simulink model "PMSM_FOC"  (R2024b)
settings: Solver=FixedStepAuto  StartTime=0.0  StopTime=0.3  FixedStep=2e-7  MaxStep=1e-6  RelTol=1e-3
model workspace (MAT data in the model file):
  Kr = 5
  Wc = 10
undefined symbols (not defined in the file): bm, J, Ld, Lq, P, Rs
libraries: simulink x2, spsDCVoltageSourceLib x1, spsMeanLib x1, slpidlib x1, spsPermanentMagnetSynchronousMachineLib x1, spsUniversalBridgeLib x1, sps_lib x1
settings Model: Creator=t'c  LastModifiedBy=t'c

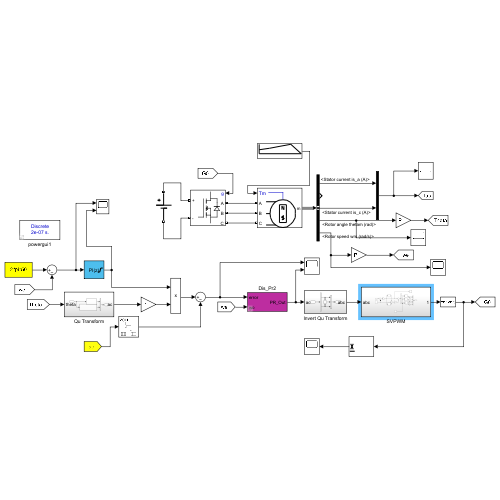
[thumbnail: Simulink's stored preview of the top-level diagram]
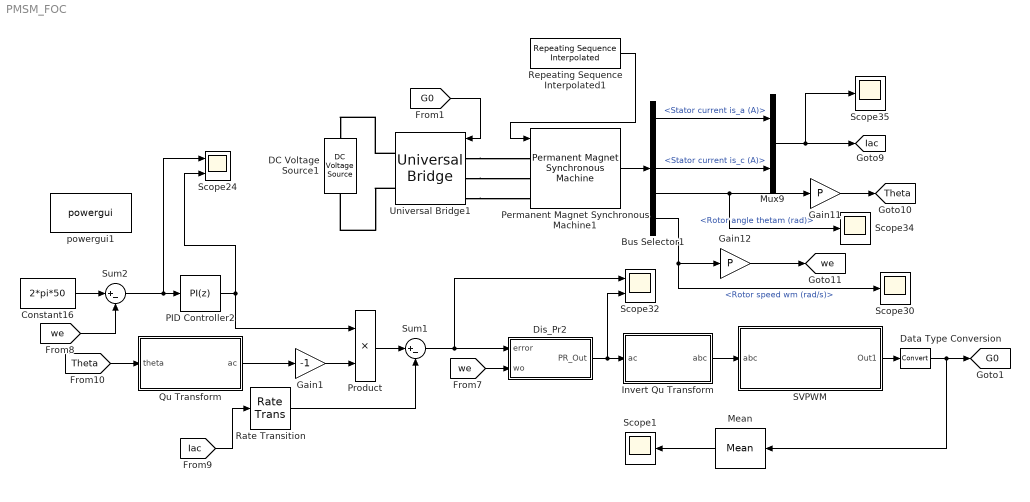
== system PMSM_FOC ==
  Bus Selector1 : BusSelector  OutputSignals=Stator current is_a (A),Stator current is_b (A),Stator current is_c (A),Rotor angle thetam (rad),Rotor speed wm (rad/s)
  Constant16 : Constant  Value=2*pi*50
  DC Voltage Source1 : spsDCVoltageSourceLib/DC Voltage Source  Amplitude=600  Measurements=None
  Data Type Conversion : DataTypeConversion  SaturateOnIntegerOverflow=off  RndMeth=Floor
  Dis_Pr2 : Subsystem  mask{Ts=5e-5, Kp=1, Kr=30, Wc=60}
      mask DialogControl pa Prompt: 参数
  Gain1 : Gain  Gain=-1
  Gain11 : Gain  Gain=P
  Gain12 : Gain  Gain=P
  Invert Qu Transform : Subsystem
  Mean : spsMeanLib/Mean  Freq=20000  Vinit=0  Ts=0
  Mux9 : Mux  Inputs=2
  PID Controller2 : slpidlib/PID Controller  Controller=PI  Form=Parallel  TimeDomain=Discrete-time  UseExternalTs=off  SampleTime=-1  IntegratorMethod=Forward Euler  FilterMethod=Forward Euler  ControllerParametersSource=internal  P=0.02  I=10  UseKiTs=off  D=0  UseExternalDerivativeSource=off  N=100  UseFilter=on  TunerSelectOption=Transfer Function Based (PID Tuner App)  InitialConditionSource=internal  InitialConditionForIntegrator=0  InitialConditionForFilter=0  DifferentiatorICPrevScaledInput=0  ExternalReset=none  TrackingMode=off  Kt=1  LimitOutput=on  SatLimitsSource=internal  UpperSaturationLimit=100  LowerSaturationLimit=-100  LinearizeAsGain=on  AntiWindupMode=none  Kb=1  LimitIntegrator=off  UpperIntegratorSaturationLimit=inf  LowerIntegratorSaturationLimit=-inf  POutMin=[]  POutMax=[]  IOutMin=[]  IOutMax=[]  DOutMin=[]  DOutMax=[]  NOutMin=[]  NOutMax=[]  SumOutMin=[]  SumOutMax=[]  SaturationOutMin=[]  SaturationOutMax=[]  PParamMin=[]  PParamMax=[]  IParamMin=[]  IParamMax=[]  DParamMin=[]  DParamMax=[]  NParamMin=[]  NParamMax=[]  KbParamMin=[]  KbParamMax=[]  KtParamMin=[]  KtParamMax=[]  KbOutMin=[]  KbOutMax=[]  KtOutMin=[]  KtOutMax=[]  IntegratorOutMin=[]  IntegratorOutMax=[]  FilterOutMin=[]  FilterOutMax=[]  SumI1OutMin=[]  SumI1OutMax=[]  SumI2OutMin=[]  SumI2OutMax=[]  SumI3OutMin=[]  SumI3OutMax=[]  SumI4OutMin=[]  SumI4OutMax=[]  SumDOutMin=[]  SumDOutMax=[]  DifferentiatorOutMin=[]  DifferentiatorOutMax=[]  FilterDiffOutCoefMin=[]  FilterDiffOutCoefMax=[]  ReciprocalOutMin=[]  ReciprocalOutMax=[]  SumDenOutMin=[]  SumDenOutMax=[]  SumNumOutMin=[]  SumNumOutMax=[]  DivideOutMin=[]  DivideOutMax=[]  UdiffTsProdOutMin=[]  UdiffTsProdOutMax=[]  NTsProdOutMin=[]  NTsProdOutMax=[]  UintegralTsProdOutMin=[]  UintegralTsProdOutMax=[]  UngainTsProdOutMin=[]  UngainTsProdOutMax=[]  ClampingZeroOutDataTypeStr=Inherit: Inherit via back propagation  ClampingZeroOutMin=[]  ClampingZeroOutMax=[]  FilterDenConstantOutDataTypeStr=Inherit: Inherit via back propagation  FilterDenConstantOutMin=[]  FilterDenConstantOutMax=[]  PCopyOutDataTypeStr=Inherit: Inherit via back propagation  PCopyOutMin=[]  PCopyOutMax=[]  NCopyOutDataTypeStr=Inherit: Inherit via back propagation  NCopyOutMin=[]  NCopyOutMax=[]  IntegratorContinuousStateAttributes=''  IntegratorStateMustResolveToSignalObject=off  IntegratorRTWStateStorageClass=Auto  FilterContinuousStateAttributes=''  FilterStateMustResolveToSignalObject=off  FilterRTWStateStorageClass=Auto  ParallelPVariant=InternalParameters  IdealPVariant=Disabled  IVariant=InternalParameters  DVariant=Disabled  IntegratorVariant=Discrete  SatVariant=Enabled  AWVariant=Passthrough  PCopyVariant=Disabled  TRVariant=Disabled  FdbkBlocksVariant=Forward  IdealPFdbkVariant=Disabled  SatFdbkVariant=Disabled  DerivativeFilterVariant=Disabled  NVariant=Disabled  NCopyVariant=Disabled_SignalSpec  FilterICVariant=Disabled  IntegratorICVariant=InternalICs  ExternalResetVariant=Disabled  TRSumVariant=Passthrough  SumFdbkVariant=Disabled  SumVariant=Sum_PI  TsampFilterVariant=InternalTs  TsampNgainVariant=Passthrough  TsampIntegralVariant=Disabled_SignalSpec  ExternalSaturationOutDataTypeStr=Inherit: Same as second input  DerivativeSourceVariant=Disabled  PreIntVariant=InternalPreInt
  Permanent Magnet Synchronous Machine1 : spsPermanentMagnetSynchronousMachineLib/Permanent Magnet Synchronous Machine  NbPhases=3  FluxDistribution=Sinusoidal  RotorType=Salient-pole  MechanicalLoad=Torque Tm  PresetModel=No  ShowDetailedParameters=on  MeasurementBus=off  Resistance=Rs  Inductance=8.5e-3  dqInductances=[Ld,Lq]  La=0.000395  MachineConstant=Flux linkage established by magnets (V.s)  Flux=flux  VoltageCst=98.6707  TorqueCst=0.816  Flat=120  Mechanical=[J bm P 0]  PolePairs=4  InitialConditions=[0,0, 0,0]  InitialConditions5ph=[0 0 0 0 0 0]  RefAngle=Aligned with phase A axis (original Park)  IterativeDiscreteModel=Trapezoidal non iterative  TsBlock=-1  TsPowergui=0
  Product : Product
  Qu Transform : Subsystem
  Rate Transition : RateTransition  OutPortSampleTime=5e-5
  Repeating Sequence Interpolated1 : simulink/Sources/Repeating Sequence Interpolated  OutValues=[0.2 0.3 0.4 0.5 0].'  TimeValues=[0 0.1 0.2 0.3 0.4 ].'  LookUpMeth=Use Input Below  tsamp=1e-1  OutMin=[]  OutMax=[]  OutDataTypeStr=double  OutputDataTypeScalingMode=double  OutDataType=fixdt(0,8)  OutScaling=2^-10
  SVPWM : Subsystem
  Scope{1,30,34..35} (4 alike) : Scope
  Scope24 : Scope  NumInputPorts=2
  Scope32 : Scope  NumInputPorts=2
  Sum1 : Sum  Inputs=|+-
  Sum2 : Sum  Inputs=|+-
  Universal Bridge1 : spsUniversalBridgeLib/Universal Bridge  Arms=3  SnubberResistance=1e5  SnubberCapacitance=inf  Device=MOSFET / Diodes  Ron=1e-3  Lon=0  ForwardVoltages="[  0  0  ]"  ForwardVoltage=0  GTOparameters=[ 10e-6 , 20e-6 ]  IGBTparameters=[ 1e-6 , 2e-6 ]  Measurements=None  Measurements_2=None  converterType=Rectifier
  powergui1 : sps_lib/powergui  Priority=1  SimulationMode=Discrete  SampleTime=2e-7  frequency=60  Iterations=50  frequencyindice=0  Pbase=100e6  ErrMax=1e-4  UnitsV=kV  UnitsW=MW  buscounter=0  FunctionMessages=off  echomessages=off  EnableUseOfTLC=off  CurrentSourceSwitches=off  DisableSnubberDevices=off  DisableRonSwitches=off  DisableVfSwitches=off  DisplayEquations=off  AutomaticDiscreteSolvers=off  SolverType=Tustin/Backward Euler (TBE)  Interpol=off  ExternalGateDelay=off  methode=off  Ts=100  x0status=blocks  SPID=on  SwTol=0  HookPort=off  NonlinearTolerance=1e-4  nMaxIteration=100  ContinueOnMaxIteration=off  RestoreLinks=warning  ResistiveCurrentMeasurement=off  Frange=[0:2:500]  Ylog=off  Xlog=on  ShowGrid=off  save=off  variable=ZData  structure=0  ZoomFFT=off  StartTime=0.0  cycles=1  DisplayStyle=1  fundamental=60  FreqAxis=off  MaxFrequency=1000  frequencyindicesteady=1  RmsSteady=1  display=off
  tag scope: G0=global, Iac=global, Theta=global, we=global
  wires:
  Repeating Sequence Interpolated1/1 -> Permanent Magnet Synchronous Machine1/1
  Sum1/1 -> Dis_Pr2/1(error), Scope32/1
  Gain12/1 -> [we]
  Gain11/1 -> [Theta]
  PID Controller2/1 -> Scope24/2, Product/1
  [we] -> Dis_Pr2/2(wo)
  Constant16/1 -> Sum2/1
  Sum2/1 -> Scope24/1, PID Controller2/1
  Mux9/1 -> [Iac], Scope35/1
  Bus Selector1/1 -> Mux9/1  "<Stator current is_a (A)>"
  Bus Selector1/4 -> Gain11/1, Scope34/1  "<Rotor angle thetam (rad)>"
  Bus Selector1/5 -> Gain12/1, Scope30/1  "<Rotor speed wm (rad/s)>"
  Permanent Magnet Synchronous Machine1/1 -> Bus Selector1/1
  Bus Selector1/3 -> Mux9/2  "<Stator current is_c (A)>"
  Dis_Pr2/1(PR_Out) -> Scope32/2, Invert Qu Transform/1(ac)
  Product/1 -> Sum1/1
  [we] -> Sum2/2
  [Iac] -> Rate Transition/1
  [G0] -> Universal Bridge1/1
  [Theta] -> Qu Transform/1(theta)
  Qu Transform/1(ac) -> Gain1/1
  Gain1/1 -> Product/2
  Mean/1 -> Scope1/1
  SVPWM/1(Out1) -> Data Type Conversion/1
  Data Type Conversion/1 -> [G0], Mean/1
  Invert Qu Transform/1(abc) -> SVPWM/1(abc)
  Rate Transition/1 -> Sum1/2
  connections:
  Universal Bridge1/LConn2 -- Permanent Magnet Synchronous Machine1/LConn2
  Universal Bridge1/LConn1 -- Permanent Magnet Synchronous Machine1/LConn1
  Universal Bridge1/RConn2 -- DC Voltage Source1/LConn1
  Universal Bridge1/RConn1 -- DC Voltage Source1/RConn1
  Universal Bridge1/LConn3 -- Permanent Magnet Synchronous Machine1/LConn3

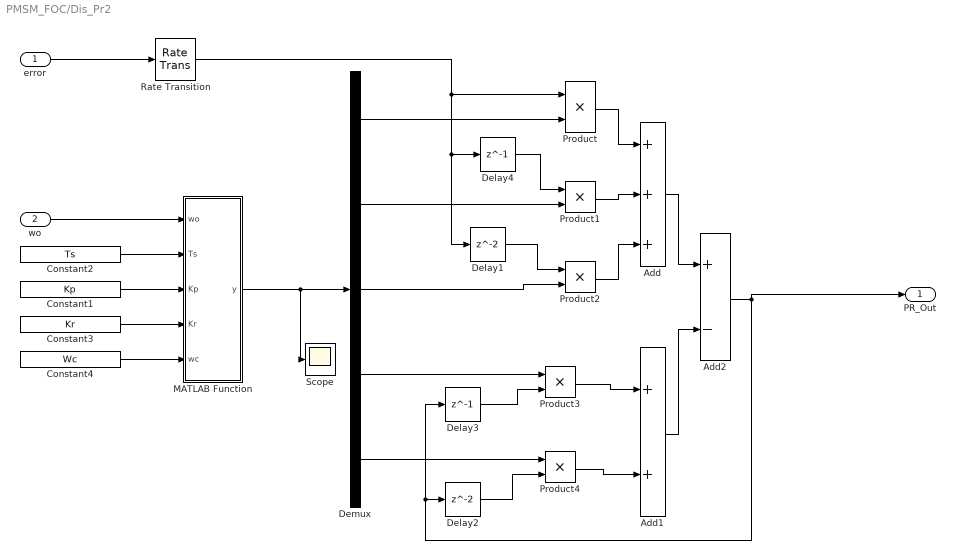
== system PMSM_FOC/Dis_Pr2 ==
  error : Inport
  wo : Inport  Port=2
  Add : Sum  Inputs=+++
  Add1 : Sum
  Add2 : Sum  Inputs=+-
  Constant1 : Constant  Value=Kp  SampleTime=-1
  Constant2 : Constant  Value=Ts  SampleTime=-1
  Constant3 : Constant  Value=Kr  SampleTime=-1
  Constant4 : Constant  Value=Wc  SampleTime=-1
  Delay1 : Delay  SampleTime=5e-5
  Delay2 : Delay  SampleTime=5e-5
  Delay3 : Delay  DelayLength=1  SampleTime=5e-5
  Delay4 : Delay  DelayLength=1  SampleTime=5e-5
  Demux : Demux  Outputs=5
  MATLAB Function : MATLAB Function  TreatAsAtomicUnit=on
  Product{,1..4} (5 alike) : Product
  Rate Transition : RateTransition  OutPortSampleTimeOpt=Inherit  OutPortSampleTime=5e-5
  Scope : Scope
  PR_Out : Outport
  wires:
  Rate Transition/1 -> Product/1, Delay4/1, Delay1/1
  Add2/1 -> PR_Out/1, Delay3/1, Delay2/1
  error/1 -> Rate Transition/1
  Constant4/1 -> MATLAB Function/5(wc)
  Constant3/1 -> MATLAB Function/4(Kr)
  Constant1/1 -> MATLAB Function/3(Kp)
  Constant2/1 -> MATLAB Function/2(Ts)
  Demux/3 -> Product2/2
  Delay1/1 -> Product2/1
  Demux/2 -> Product1/2
  Delay4/1 -> Product1/1
  Product/1 -> Add/1
  Product1/1 -> Add/2
  Product2/1 -> Add/3
  Product3/1 -> Add1/1
  Product4/1 -> Add1/2
  Add/1 -> Add2/1
  Add1/1 -> Add2/2
  Delay2/1 -> Product4/2
  wo/1 -> MATLAB Function/1(wo)
  Delay3/1 -> Product3/2
  Demux/4 -> Product3/1
  Demux/5 -> Product4/1
  Demux/1 -> Product/2
  MATLAB Function/1(y) -> Demux/1, Scope/1

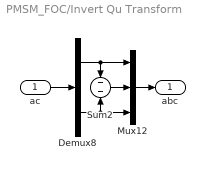
== system PMSM_FOC/Invert Qu Transform ==
  ac : Inport
  Demux8 : Demux  Outputs=2
  Mux12 : Mux  Inputs=3
  Sum2 : Sum  Inputs=-|-
  abc : Outport
  wires:
  Demux8/1 -> Mux12/1, Sum2/1
  ac/1 -> Demux8/1
  Sum2/1 -> Mux12/2
  Demux8/2 -> Mux12/3, Sum2/2
  Mux12/1 -> abc/1

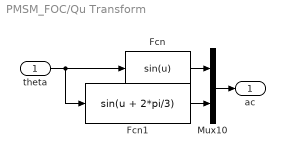
== system PMSM_FOC/Qu Transform ==
  theta : Inport
  Fcn : Fcn  Expr=sin(u)
  Fcn1 : Fcn  Expr=sin(u + 2*pi/3)
  Mux10 : Mux  Inputs=2
  ac : Outport
  wires:
  Mux10/1 -> ac/1
  Fcn/1 -> Mux10/1
  Fcn1/1 -> Mux10/2
  theta/1 -> Fcn1/1, Fcn/1

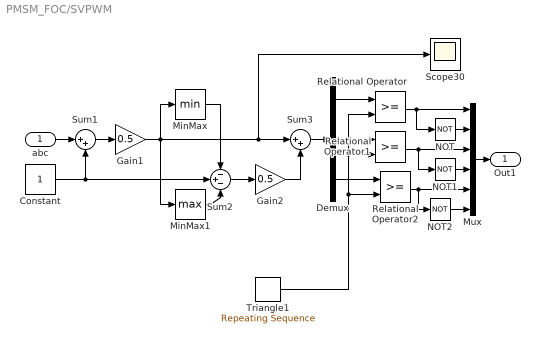
== system PMSM_FOC/SVPWM ==
  abc : Inport
  Constant : Constant
  Demux : Demux  Outputs=3
  Gain1 : Gain  Gain=0.5
  Gain2 : Gain  Gain=0.5
  MinMax : MinMax
  MinMax1 : MinMax  Function=max
  Mux : Mux  Inputs=6
  NOT : Logic  Operator=NOT  IconShape=distinctive  AllPortsSameDT=off  OutDataTypeStr=boolean
  NOT1 : Logic  Operator=NOT  IconShape=distinctive  AllPortsSameDT=off  OutDataTypeStr=boolean
  NOT2 : Logic  Operator=NOT  IconShape=distinctive  AllPortsSameDT=off  OutDataTypeStr=boolean
  Relational Operator : RelationalOperator  OutDataTypeStr=boolean  RndMeth=Simplest  InputSameDT=off
  Relational Operator1 : RelationalOperator  OutDataTypeStr=boolean  RndMeth=Simplest  InputSameDT=off
  Relational Operator2 : RelationalOperator  OutDataTypeStr=boolean  RndMeth=Simplest  InputSameDT=off
  Scope30 : Scope
  Sum1 : Sum  Inputs=|++
  Sum2 : Sum  Inputs=-+-
  Sum3 : Sum  Inputs=|++
  Triangle1 : simulink/Sources/Repeating Sequence  rep_seq_t=[0 1/20000/2 1/20000]  rep_seq_y=[0 1 0]
  Out1 : Outport
  wires:
  abc/1 -> Sum1/1
  Sum1/1 -> Gain1/1
  Constant/1 -> Sum1/2, Sum2/2
  MinMax/1 -> Sum2/1
  Gain1/1 -> Scope30/1, Sum3/1, MinMax1/1, MinMax/1
  MinMax1/1 -> Sum2/3
  Sum2/1 -> Gain2/1
  Gain2/1 -> Sum3/2
  Sum3/1 -> Demux/1
  Demux/2 -> Relational Operator1/1
  Demux/1 -> Relational Operator/1
  Demux/3 -> Relational Operator2/1
  Triangle1/1 -> Relational Operator/2, Relational Operator1/2, Relational Operator2/2
  NOT/1 -> Mux/2
  Relational Operator/1 -> NOT/1, Mux/1
  Relational Operator1/1 -> NOT1/1, Mux/3
  Relational Operator2/1 -> NOT2/1, Mux/5
  NOT1/1 -> Mux/4
  NOT2/1 -> Mux/6
  Mux/1 -> Out1/1

== matlab function PMSM_FOC/Dis_Pr2/MATLAB Function ==
  settings: sampleTime=1e
  data: wo input; y output; Ts input; Kp input; Kr input; wc input
function y = fcn( wo,Ts,Kp,Kr,wc)
temp = 4 / Ts / Ts + 4 * wc / Ts + wo * wo;
B0 = (4 * Kp / Ts / Ts + 4 * wc * (Kp + Kr) / Ts+ Kp * wo * wo) / temp;
B1 = (-8 * Kp / Ts / Ts + 2 * Kp * wo * wo) / temp;
B2 = (4 * Kp / Ts / Ts - 4 * wc / Ts * (Kp + Kr) + Kp * wo * wo) / temp;
A1 = (-8 / Ts / Ts + 2 * wo * wo) / temp;
A2 = (4 / Ts / Ts - 4 * wc / Ts + wo * wo) / temp;
y = [B0;B1;B2;A1;A2];
